simulink model "DIGITAL_WATCH_STAGE6"  (R2026b)
settings: Solver=VariableStepAuto  StopTime=125
libraries: simulink_extras x14
settings Model: Creator=Trealer  LastModifiedBy=Trealer

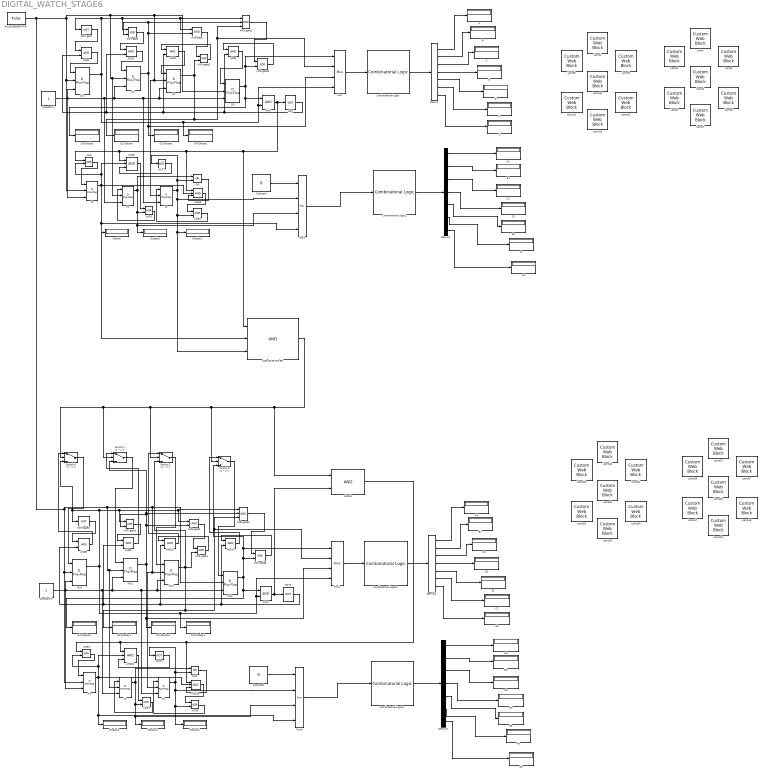
== system DIGITAL_WATCH_STAGE6 ==
  A{,1..3} (4 alike) : Display
  AND{,1..4,8..11,14} (10 alike) : Logic  IconShape=distinctive  AllPortsSameDT=off  OutDataTypeStr=boolean
  "AND-GATE MIN-EN " : Logic  Inputs=3  IconShape=distinctive  AllPortsSameDT=off  OutDataTypeStr=boolean
  AND-gate : Logic  IconShape=distinctive  AllPortsSameDT=off  OutDataTypeStr=boolean
  AND-gate1 : Logic  IconShape=distinctive  AllPortsSameDT=off  OutDataTypeStr=boolean
  AND-gate2 : Logic  Inputs=3  IconShape=distinctive  AllPortsSameDT=off  OutDataTypeStr=boolean
  AND-gate3 : Logic  Inputs=3  IconShape=distinctive  AllPortsSameDT=off  OutDataTypeStr=boolean
  AND{5..6,12..13} (4 alike) : Logic  Inputs=3  IconShape=distinctive  AllPortsSameDT=off  OutDataTypeStr=boolean
  B{,1..3} (4 alike) : Display
  C{,1..3} (4 alike) : Display
  CMU : Logic  IconShape=distinctive  AllPortsSameDT=off  OutDataTypeStr=boolean
  Combinatorial Logic : CombinatorialLogic  TruthTable=|
      | [
      | 1 1 1 1 1 1 0;
      | 0 1 1 0 0 0 0;
      | 1 1 0 1 1 0 1;
      | 1 1 1 1 0 0 1;
      | 0 1 1 0 0 1 1;
      | 1 0 1 1 0 1 1;
      | 1 0 1 1 1 1 1;
      | 1 1 1 0 0 0 0;
      | 1 1 1 1 1 1 1;
      | 1 1 1 1 0 1 1;
      | 0 0 0 0 0 0 0;
      | 0 0 0 0 0 0 0;
      | 0 0 0 0 0 0 0;
      | 0 0 0 0 0 0 0;
      | 0 0 0 0 0 0 0;
      | 0 0 0 0 0 0 0
      | ]
  Combinatorial Logic1 : CombinatorialLogic  TruthTable=|
      | [
      | 1 1 1 1 1 1 0;
      | 0 1 1 0 0 0 0;
      | 1 1 0 1 1 0 1;
      | 1 1 1 1 0 0 1;
      | 0 1 1 0 0 1 1;
      | 1 0 1 1 0 1 1;
      | 1 0 1 1 1 1 1;
      | 1 1 1 0 0 0 0;
      | 1 1 1 1 1 1 1;
      | 1 1 1 1 0 1 1;
      | 0 0 0 0 0 0 0;
      | 0 0 0 0 0 0 0;
      | 0 0 0 0 0 0 0;
      | 0 0 0 0 0 0 0;
      | 0 0 0 0 0 0 0;
      | 0 0 0 0 0 0 0
      | ]
  Combinatorial Logic2 : CombinatorialLogic  TruthTable=|
      | [
      | 1 1 1 1 1 1 0;
      | 0 1 1 0 0 0 0;
      | 1 1 0 1 1 0 1;
      | 1 1 1 1 0 0 1;
      | 0 1 1 0 0 1 1;
      | 1 0 1 1 0 1 1;
      | 1 0 1 1 1 1 1;
      | 1 1 1 0 0 0 0;
      | 1 1 1 1 1 1 1;
      | 1 1 1 1 0 1 1;
      | 0 0 0 0 0 0 0;
      | 0 0 0 0 0 0 0;
      | 0 0 0 0 0 0 0;
      | 0 0 0 0 0 0 0;
      | 0 0 0 0 0 0 0;
      | 0 0 0 0 0 0 0
      | ]
  Combinatorial Logic3 : CombinatorialLogic  TruthTable=|
      | [
      | 1 1 1 1 1 1 0;
      | 0 1 1 0 0 0 0;
      | 1 1 0 1 1 0 1;
      | 1 1 1 1 0 0 1;
      | 0 1 1 0 0 1 1;
      | 1 0 1 1 0 1 1;
      | 1 0 1 1 1 1 1;
      | 1 1 1 0 0 0 0;
      | 1 1 1 1 1 1 1;
      | 1 1 1 1 0 1 1;
      | 0 0 0 0 0 0 0;
      | 0 0 0 0 0 0 0;
      | 0 0 0 0 0 0 0;
      | 0 0 0 0 0 0 0;
      | 0 0 0 0 0 0 0;
      | 0 0 0 0 0 0 0
      | ]
  Constant : Constant  Value=0  OutDataTypeStr=boolean
  Constant 1 : Constant  OutDataTypeStr=boolean
  Constant 2 : Constant  OutDataTypeStr=boolean
  Constant1 : Constant  Value=0  OutDataTypeStr=boolean
  D{,1..3} (4 alike) : Display
  Demux{,1..3} (4 alike) : Demux  Outputs=7
  Display{,1..5} (6 alike) : Display
  E{,1..3} (4 alike) : Display
  F{,1..3} (4 alike) : Display
  G{,1..3} (4 alike) : Display
  Lamp{,1..27} (28 alike) : CustomWebBlock  LabelPosition=Hide  ShowInitialText=on  Configuration="{\"components\":[{\"name\":\"BackgroundImageComponent\",\"settings\":{\"image\":{\"size\":[150,150],\"src\":\"data:image\\/svg+xml;base64,PHN2ZyB4bWxucz0iaHR0cDovL3d3dy53My5vcmcvMjAwMC9zdmciIHhtbG5zOnhsaW5rPSJodHRwOi8vd3d3LnczLm9yZy8xOTk5L3hsaW5rIiB2aWV3Qm94PSIwIDAgNTAwIDUwMCI+PGRlZnM+PHN0eWxlPi5he2ZpbGw6dXJsKCNhKTt9LmJ7ZmlsbDp1cmwoI2IpO30uY3tmaWxsOnVybCgjYyk7fTwvc3R5bGU+PHJhZGlhbEdyYWRpZW50IGlkPSJhIiBjeD0iMjgzLjg0IiBjeT0iLTQ2Ni4zNyIgcj0iMzc1Ljc1IiBncmFkaWVudFRyYW5zZm9ybT0ibWF0cml4KDEuMzksIDAsIDAsIC0xLjM5LCAtMTUzLjU2LCAtNjQ0LjA4KSIg ...(+2088 chars)\",\"srcOrientation\":\"Right\"},\"position\":[0,0,1,1],\"scaleMode\":\"0\"}},{\"name\":\"LampStateComponent\",\"settings\":{\"position\":[0,0,1,1],\"states\":[{\"icon\":{\"customSrc\":\"data:image\\/svg+xml;base64,PHN2ZyBpZD0iTGF5ZXJfMSIgZGF0YS1uYW1lPSJMYXllciAxIiB4bWxucz0iaHR0cDovL3d3dy53My5vcmcvMjAwMC9zdmciIHZpZXdCb3g9IjAgMCA0MTEgNDU4Ij48ZGVmcz48c3R5bGU+LmNscy0xe2ZpbGw6I2ZkZjhjMTt9LmNscy0ye2ZpbGw6I2ZlZTEwMDt9LmNscy0ze2ZpbGw6IzIzMWYyMDt9LmNscy00e2ZpbGw6I2EwOWY5Zjt9LmNscy00LC5jbHMtNSwuY2xzLTZ7c3Ryb2tlOiMyMzFmMjA7c3Ryb2tlLW1pdGVybGltaXQ6MTA7fS5jbHMtNXtmaWxsOiNmZmY7fS5jbHMtNntmaWxsOm5vbmU7fTwvc3R5bGU+PC9kZWZz ...(+5168 chars)\",\"id\":-1,\"srcOrientation\":\"Right\",\"type\":\"custom\"},\"iconScale\":0.8,\"metadata\":{},\"overlayType\":\"intersect\",\"shape\":{\"color\":[0.725,0,0],\"opacity\":1,\"position\":[0.1,0.1,0.8,0.8],\"type\":\"ellipse\"},\"value\":[]},{\"icon\":{\"customSrc\":\"data:image\\/svg+xml;base64,PHN2ZyBpZD0iTGF5ZXJfMSIgZGF0YS1uYW1lPSJMYXllciAxIiB4bWxucz0iaHR0cDovL3d3dy53My5vcmcvMjAwMC9zdmciIHZpZXdCb3g9IjAgMCA0MTEgNDU4Ij48ZGVmcz48c3R5bGU+LmNscy0xe2ZpbGw6I2ZkZjhjMTt9LmNscy0ye2ZpbGw6I2ZlZTEwMDt9LmNscy0ze2ZpbGw6IzIzMWYyMDt9LmNscy00e2ZpbGw6I2EwOWY5Zjt9LmNscy00LC5jbHMtNSwuY2xzLTZ7c3Ryb2tlOiMyMzFmMjA7c3Ryb2tlLW1pdGVybGltaXQ6MTA7fS5jbHMtNXtmaWxsOiNmZmY7fS5jbHMtNntmaWxsOm5vbmU7fTwvc3R5bGU+PC9kZWZz ...(+5168 chars)\",\"id\":-1,\"srcOrientation\":\"Right\",\"type\":\"custom\"},\"iconScale\":0.8,\"metadata\":{\"useDefaults\":{\"customIcon\":true,\"icon\":true,\"overlayType\":true,\"shape\":true,\"sizeAndPosition\":true}},\"overlayType\":\"intersect\",\"shape\":{\"color\":[0,0,0],\"opacity\":1,\"position\":[0.1,0.1,0.8,0.8],\"type\":\"ellipse\"},\"value\":\"0\"},{\"icon\":{\"customSrc\":\"data:image\\/svg+xml;base64,PHN2ZyBpZD0iTGF5ZXJfMSIgZGF0YS1uYW1lPSJMYXllciAxIiB4bWxucz0iaHR0cDovL3d3dy53My5vcmcvMjAwMC9zdmciIHZpZXdCb3g9IjAgMCA0MTEgNDU4Ij48ZGVmcz48c3R5bGU+LmNscy0xe2ZpbGw6I2ZkZjhjMTt9LmNscy0ye2ZpbGw6I2ZlZTEwMDt9LmNscy0ze2ZpbGw6IzIzMWYyMDt9LmNscy00e2ZpbGw6I2EwOWY5Zjt9LmNscy00LC5jbHMtNSwuY2xzLTZ7c3Ryb2tlOiMyMzFmMjA7c3Ryb2tlLW1pdGVybGltaXQ6MTA7fS5jbHMtNXtmaWxsOiNmZmY7fS5jbHMtNntmaWxsOm5vbmU7fTwvc3R5bGU+PC9kZWZz ...(+5168 chars)\",\"id\":-1,\"srcOrientation\":\"Right\",\"type\":\"custom\"},\"iconScale\":0.8,\"metadata\":{\"useDefaults\":{\"customIcon\":true,\"icon\":true,\"overlayType\":true,\"shape\":true,\"sizeAndPosition\":true}},\"overlayType\":\"intersect\",\"shape\":{\"color\":[0,1,0],\"opacity\":1,\"position\":[0.1,0.1,0.8,0.8],\"type\":\"ellipse\"},\"value\":\"1\"}],\"valueType\":\"discrete\"}},{\"name\":\"ForegroundImageComponent\",\"settings\":{\"image\":{\"size\":[150,150],\"src\":\"data:image\\/svg+xml;base64,PHN2ZyB4bWxucz0iaHR0cDovL3d3dy53My5vcmcvMjAwMC9zdmciIHhtbG5zOnhsaW5rPSJodHRwOi8vd3d3LnczLm9yZy8xOTk5L3hsaW5rIiB2aWV3Qm94PSIwIDAgNTAwIDUwMCI+PGRlZnM+PHN0eWxlPi5he2ZpbGw6dXJsKCNhKTt9PC9zdHlsZT48bGluZWFyR3JhZGllbnQgaWQ9ImEiIHgxPSIxNzMuMDUiIHkxPSItNjI3Ljc4IiB4Mj0iMTczLjA1IiB5Mj0iLTUyMi40MyIgZ3JhZGllbnRUcmFuc2Zvcm09Im1hdHJpeCgxLjI5LCAwLCAwLCAtMS4zMywgMjcuMTMsIC02MjguMzEpIiBncmFkaWVudFVuaXRzPSJ1c2VyU3BhY2VPblVzZSI+PHN0b3Agb2Zmc2V0PSIwIiBzdG9wLWNvbG9yPSIjZmZmIiBzdG9wLW9wYWNpdHk9IjAuMjUiLz48c3RvcCBvZmZzZXQ9IjEiIHN0b3AtY29sb3I9IiNmZmYiIHN0b3Atb3BhY2l0eT0iMCIvPjwvbGluZWFyR3JhZGllbnQ+PC9kZWZzPjxwYXRoIGNsYXNzPSJhIiBkPSJNNDI5LjMsMTkwLjY2QzQwMi40NSwxMTQuNTEsMzMyLjY3LDYwLjE3LDI1MC44NSw2MC4xN2MtODMuNDMsMC0xNTQuMjgsNTYuNDItMTc5Ljk1LDEzNSwxNS4zNCwzOSw4OC4xMSw3LDE3Ny4wNyw3QzM0MCwyMDIuMDgsNDE3LjI2LDIzNi40Niw0MjkuMywxOTAuNjZaIi8+PC9zdmc+\",\"srcOrientation\":\"Right\"},\"isForeground\":1,\"position\":[0,0,1,1],\"scaleMode\":\"0\"}}],\"derived\":{\"blockParameters\":{\"CustomIcon\":\"data:image\\/svg+xml;base64,PHN2ZyBpZD0iTGF5ZXJfMSIgZGF0YS1uYW1lPSJMYXllciAxIiB4bWxucz0iaHR0cDovL3d3dy53My5vcmcvMjAwMC9zdmciIHZpZXdCb3g9IjAgMCA0MTEgNDU4Ij48ZGVmcz48c3R5bGU+LmNscy0xe2ZpbGw6I2ZkZjhjMTt9LmNscy0ye2ZpbGw6I2ZlZTEwMDt9LmNscy0ze2ZpbGw6IzIzMWYyMDt9LmNscy00e2ZpbGw6I2EwOWY5Zjt9LmNscy00LC5jbHMtNSwuY2xzLTZ7c3Ryb2tlOiMyMzFmMjA7c3Ryb2tlLW1pdGVybGltaXQ6MTA7fS5jbHMtNXtmaWxsOiNmZmY7fS5jbHMtNntmaWxsOm5vbmU7fTwvc3R5bGU+PC9kZWZz ...(+5168 chars)\",\"DefaultColor\":[0.725,0,0],\"Icon\":\"Custom\",\"StateColors\":[{\"color\":[0,0,0],\"value\":\"0\"},{\"color\":[0,1,0],\"value\":\"1\"}],\"StateValueType\":\"discrete\",\"fixedAspectRatio\":\"on\"}},\"settings\":{\"BindingType\":\"signal\",\"aspectRatio\":1.032258064516129,\"backgroundColor\":[0,0,0],\"backgroundOffset\":0.14,\"backgroundOpacity\":1,\"blockOrientation\":\"Right\",\"fixedAspectRatio\":\"on\",\"showBackgroundColor\":false,\"value\":0,\"version\":\"R2023a\"},\"type\":\"Lamp\"}"
  MU{0..3} (4 alike) : simulink_extras/Flip Flops/D Flip-Flop
  Mux{,1..3} (4 alike) : Mux
  NOT{,1..3} (4 alike) : Logic  Operator=NOT  IconShape=distinctive  AllPortsSameDT=off  OutDataTypeStr=boolean
  NOT-gate : Logic  Operator=NOT  IconShape=distinctive  AllPortsSameDT=off  OutDataTypeStr=boolean
  NOT-gate1 : Logic  Operator=NOT  IconShape=distinctive  AllPortsSameDT=off  OutDataTypeStr=boolean
  OR : Logic  Operator=OR  IconShape=distinctive  AllPortsSameDT=off  OutDataTypeStr=boolean
  OR1 : Logic  Operator=OR  IconShape=distinctive  AllPortsSameDT=off  OutDataTypeStr=boolean
  PULSE GENERATOR : DiscretePulseGenerator  PulseType=Time based  Period=1  PulseWidth=50
  Q{0..3} (4 alike) : simulink_extras/Flip Flops/D Flip-Flop
  Q0-Display : Display
  Q0-Display1 : Display
  Q1-Display : Display
  Q1-Display1 : Display
  Q2-Display : Display
  Q2-Display1 : Display
  Q3-Display : Display
  Q3-Display1 : Display
  Switch-{0..3} (4 alike) : Switch  Criteria=u2 ~= 0  SaturateOnIntegerOverflow=off  InputSameDT=off
  T{0..5} (6 alike) : simulink_extras/Flip Flops/D Flip-Flop
  XOR{,1..5} (6 alike) : Logic  Operator=XOR  IconShape=distinctive  AllPortsSameDT=off  OutDataTypeStr=boolean
  XOR-gate{,1..5} (6 alike) : Logic  Operator=XOR  IconShape=distinctive  AllPortsSameDT=off  OutDataTypeStr=boolean
  wires:
  Constant 1/1 -> T1/3, T2/3, Q3/3, Q2/3, Q1/3, Q0/3, T0/3
  Q0/1 -> Mux/4, AND/2, Q0-Display/1, AND-gate/1, AND-gate2/1, XOR-gate/1, NOT-gate/1
  Q1/1 -> Mux/3, Q1-Display/1, AND-gate2/2, XOR-gate/2, AND-gate/2
  AND-gate/1 -> XOR-gate2/1
  Q2/1 -> Mux/2, AND-gate2/3, Q2-Display/1, XOR-gate2/2
  AND-gate2/1 -> XOR-gate3/1
  Q3/1 -> XOR-gate3/2, Mux/1, Q3-Display/1, AND/1
  AND/1 -> "AND-GATE MIN-EN "/1, AND6/1, AND5/1, XOR/1, NOT/1
  NOT-gate/1 -> AND1/1
  XOR-gate/1 -> AND2/1
  XOR-gate2/1 -> AND3/1
  XOR-gate3/1 -> AND4/1
  AND1/1 -> Q0/1
  AND2/1 -> Q1/1
  AND3/1 -> Q2/1
  AND4/1 -> Q3/1
  NOT/1 -> AND4/2, AND3/2, AND1/2, AND2/2
  T0/1 -> Display/1, Mux1/4, "AND-GATE MIN-EN "/2, AND6/2, AND5/2, XOR/2
  XOR/1 -> T0/1
  T2/1 -> "AND-GATE MIN-EN "/3, Display2/1, XOR2/2, Mux1/2, OR/2, NOT1/1
  NOT1/1 -> AND5/3
  AND5/1 -> XOR1/1
  T1/1 -> Mux1/3, Display1/1, XOR1/2, OR/1
  OR/1 -> AND6/3
  AND6/1 -> XOR2/1
  XOR1/1 -> T1/1
  XOR2/1 -> T2/1
  Mux/1 -> Combinatorial Logic/1
  Combinatorial Logic/1 -> Demux/1
  Demux/1 -> A/1
  Demux/2 -> B/1
  Demux/3 -> C/1
  Demux/4 -> D/1
  Demux/5 -> E/1
  Demux/6 -> F/1
  Demux/7 -> G/1
  Combinatorial Logic1/1 -> Demux1/1
  Constant/1 -> Mux1/1
  Mux1/1 -> Combinatorial Logic1/1
  Demux1/2 -> B1/1
  Demux1/6 -> F1/1
  Demux1/1 -> A1/1
  Demux1/7 -> G1/1
  Demux1/4 -> D1/1
  Demux1/3 -> C1/1
  Demux1/5 -> E1/1
  Demux3/2 -> B3/1
  Demux3/4 -> D3/1
  Demux3/3 -> C3/1
  Demux3/7 -> G3/1
  Constant1/1 -> Mux3/1
  Demux3/5 -> E3/1
  Demux3/1 -> A3/1
  Combinatorial Logic3/1 -> Demux3/1
  PULSE GENERATOR/1 -> MU3/2, T5/2, MU2/2, MU1/2, T4/2, MU0/2, T3/2, Q3/2, T2/2, Q2/2, Q1/2, T1/2, Q0/2, T0/2
  MU3/1 -> Switch-3/3, Mux2/1, XOR-gate5/2, Q3-Display1/1, CMU/1
  XOR-gate1/1 -> AND9/1
  NOT-gate1/1 -> AND8/1
  Demux2/3 -> C2/1
  XOR-gate4/1 -> AND10/1
  CMU/1 -> AND14/2, NOT2/1
  NOT3/1 -> AND12/3
  XOR5/1 -> T5/1
  XOR3/1 -> T3/1
  MU2/1 -> XOR-gate4/2, Mux2/2, AND-gate3/3, Q2-Display1/1, Switch-2/3
  AND-gate1/1 -> XOR-gate4/1
  XOR-gate5/1 -> AND11/1
  Demux2/2 -> B2/1
  Demux2/1 -> A2/1
  Combinatorial Logic2/1 -> Demux2/1
  Demux2/7 -> G2/1
  OR1/1 -> AND13/3
  MU0/1 -> AND-gate1/1, AND-gate3/1, XOR-gate1/1, Switch-0/3, NOT-gate1/1, Mux2/4, CMU/2, Q0-Display1/1
  NOT2/1 -> AND11/2, AND10/2, AND8/2, AND9/2
  Constant 2/1 -> T4/3, T5/3, MU3/3, MU2/3, MU1/3, MU0/3, T3/3
  Demux2/4 -> D2/1
  MU1/1 -> Switch-1/3, AND-gate3/2, XOR-gate1/2, AND-gate1/2, Mux2/3, Q1-Display1/1
  Demux2/5 -> E2/1
  Mux3/1 -> Combinatorial Logic3/1
  Demux2/6 -> F2/1
  AND13/1 -> XOR5/1
  T3/1 -> Display3/1, Mux3/4, AND12/2, XOR3/2, AND13/2
  AND-gate3/1 -> XOR-gate5/1
  AND12/1 -> XOR4/1
  XOR4/1 -> T4/1
  Mux2/1 -> Combinatorial Logic2/1
  T5/1 -> Display5/1, XOR5/2, Mux3/2, OR1/2, NOT3/1
  Demux3/6 -> F3/1
  T4/1 -> Mux3/3, Display4/1, XOR4/2, OR1/1
  "AND-GATE MIN-EN "/1 -> AND14/1, Switch-3/2, Switch-2/2, Switch-1/2, Switch-0/2
  AND8/1 -> Switch-0/1
  Switch-0/1 -> MU0/1
  AND9/1 -> Switch-1/1
  Switch-1/1 -> MU1/1
  AND10/1 -> Switch-2/1
  Switch-2/1 -> MU2/1
  AND11/1 -> Switch-3/1
  Switch-3/1 -> MU3/1
  AND14/1 -> AND13/1, AND12/1, XOR3/1
